simulink model "cooling_loop"  (R2026b)
settings: Solver=ode4  StartTime=0  StopTime=1726  FixedStep=0.10000000000000001
model workspace (MAT data in the model file):
  C = 30000
  T0 = 85
  T_amb = 31
  cyc_Qin = [2000 2000 2000 2000 2000 2000 2000 2000 2000 2000 2000 2000 ... (17261 elements, 1x17261)]
  cyc_mdot = [2.23596170404 2.23596170404 2.23596170404 2.23596170404 2.23596170404 2.23596170404 2.23596170404 2.23596170404 2.23596170404 2.23596170404 2.23596170404 2.23596170404 ... (17261 elements, 1x17261)]
  cyc_t = [0 0.1 0.2 0.3 0.4 0.5 0.6 0.7 0.8 0.9 1 1.1 ... (17261 elements, 1x17261)]
  cyc_v = [0 0 0 0 0 0 0 0 0 0 0 0 ... (17261 elements, 1x17261)]
  dt = 0.1
  eta_ram = 0.3
  fan_cfm = 300
  fan_off = 90
  fan_on = 95
  hA_ext = 10
  thermo_full = 95
  thermo_min = 0.02
  thermo_open = 82
(part 2 of 2)

== matlab function cooling_loop/Radiator and fan ==
  data: u input; y output
function y = radiator_and_fan(u)
%#codegen
% u = [coolant temperature; coolant flow through the radiator; fan on;
%      car speed; ram-air share; fan airflow (CFM); air temperature]
% y = [heat to the air (W); air speed at the core face (m/s)]
% The equations are in ../matlab/radiator_block.m, shared with the scripts.
y = radiator_block(u);
